simulink model "tire_pressure_demo"  (R2026b)
settings: Solver=VariableStepAuto  StopTime=60
settings Model: DataDictionary=tire_pressure_demo.sldd  Creator=SET6KOR  LastModifiedBy=SET6KOR

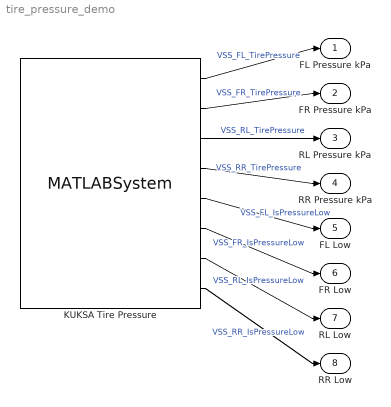
== system tire_pressure_demo ==
  KUKSA Tire Pressure : MATLABSystem  System=TirePressureSystem  Host=127.0.0.1  Port=55556  Timeout=1.0  SampleTime=1.0  PressureDropPerSecond=1  LowPressureThreshold=210  AllowInsecureRemote=false
      mask Type: TirePressureSystem
  FL Pressure kPa : Outport
  FR Pressure kPa : Outport  Port=2
  RL Pressure kPa : Outport  Port=3
  RR Pressure kPa : Outport  Port=4
  FL Low : Outport  Port=5
  FR Low : Outport  Port=6
  RL Low : Outport  Port=7
  RR Low : Outport  Port=8
  wires:
  KUKSA Tire Pressure/1 -> FL Pressure kPa/1  "VSS_FL_TirePressure"
  KUKSA Tire Pressure/2 -> FR Pressure kPa/1  "VSS_FR_TirePressure"
  KUKSA Tire Pressure/3 -> RL Pressure kPa/1  "VSS_RL_TirePressure"
  KUKSA Tire Pressure/4 -> RR Pressure kPa/1  "VSS_RR_TirePressure"
  KUKSA Tire Pressure/5 -> FL Low/1  "VSS_FL_IsPressureLow"
  KUKSA Tire Pressure/6 -> FR Low/1  "VSS_FR_IsPressureLow"
  KUKSA Tire Pressure/7 -> RL Low/1  "VSS_RL_IsPressureLow"
  KUKSA Tire Pressure/8 -> RR Low/1  "VSS_RR_IsPressureLow"
